simulink model "MATE_2level_DriveOversampling"  (R2024b)
settings: Solver=FixedStepDiscrete  StartTime=0.0  StopTime=1  FixedStep=Ts  MaxStep=10e-6  RelTol=1e-3
PostLoadFcn:
  | Ts=2e-6; Ts_Power=30e-6;
InitFcn:
  | Ts=2e-6; Ts_Power=30e-6;
libraries: simetranss x10, nesl_utility x9, fl_lib x6, ee_lib x6, batteryecm_lib x2, simulink x1
settings Model: ARTEMISmethode_block_infos=$$__separator__$$  ModifiedByFormat=x  Creator=Kyle  LastModifiedBy=x
settings SolverCC: AlgebraicLoopSolver=TrustRegion
settings DataIOCC: SaveFormat=Array  SignalLoggingSaveFormat=ModelDataLogs  SaveOutput=off  SignalLogging=off  SaveTime=off  ReturnWorkspaceOutputs=off
settings OptimizationCC: OptimizeBlockIOStorage=off  BufferReuse=off  GlobalBufferReuse=off  ExpressionFolding=off  ExpressionDepthLimit=2147483647  LocalBlockOutputs=off  InitFltsAndDblsToZero=on  LifeSpan=inf
settings DebuggingCC: SaveWithParameterizedLinksMsg=none  UnderspecifiedInitializationDetection=Classic  MergeDetectMultiDrivingBlocksExec=none  SignalResolutionControl=TryResolveAllWithWarning  SolverPrmCheckMsg=warning  MultiTaskDSMMsg=warning  MultiTaskCondExecSysMsg=none  FcnCallInpInsideContextMsg=warning  UnconnectedInputMsg=warning  UnconnectedOutputMsg=warning  UnconnectedLineMsg=warning  AllowSymbolicDim=off  StateNameClashWarn=warning  SFUnexpectedBacktrackingDiag=warning  SFNoUnconditionalDefaultTransitionDiag=warning  SFExecutionAtInitializationDiag=none  ArithmeticOperatorsInVariantConditions=warning
settings HardwareCC: ProdBitPerPointer=32  ProdBitPerSizeT=32  ProdBitPerPtrDiffT=32  ProdLargestAtomicFloat=None  ProdIntDivRoundTo=Undefined  ProdEndianess=Unspecified  ProdWordSize=32  ProdHWDeviceType=32-bit Generic  TargetHWDeviceType=32-bit Generic
settings ModelReferenceCC: EnableRefExpFcnMdlSchedulingChecks=on  PropagateSignalLabelsOutOfModel=off
settings SFSimCC: SimUseLocalCustomCode=off  CustomCodeUndefinedFunction=UseInterfaceOnly
settings RTWCC: RTWUseLocalCustomCode=off  GPUComputeCapability=3.5
settings CodeAppCC: StateflowObjectComments=on
settings GRTTargetCC: TargetFcnLib=ansi_tfl_tmw.mat  TargetLangStandard=C89/C90 (ANSI)  CombineOutputUpdateFcns=off  GRTInterface=on
settings ConfigComp: CovMetricSettings=dw  CovSaveCumulativeToWorkspaceVar=on  CovSaveSingleToWorkspaceVar=on  CovExternalEMLEnable=off
settings SimscapeCC: SimscapeNormalizeSystem=off

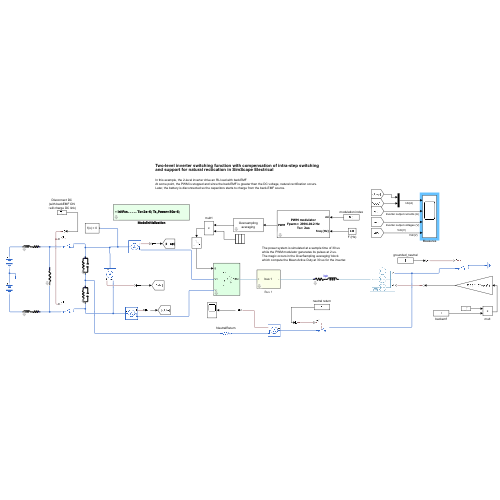
[thumbnail: Simulink's stored preview of the top-level diagram]
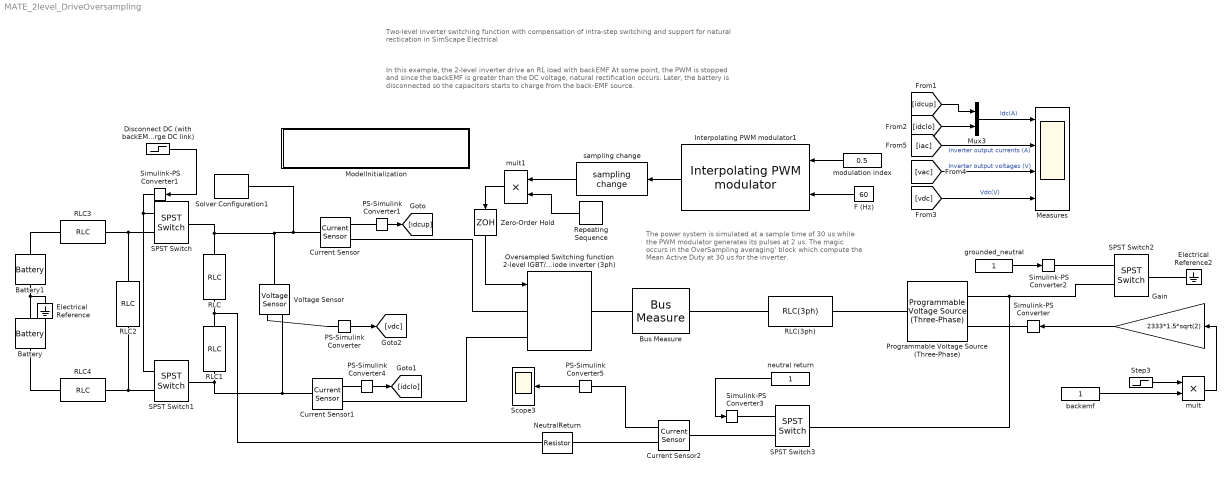
== system MATE_2level_DriveOversampling ==
  note: The power system is simulated at a sample time of 30 us
      | while the PWM modulator generates its pulses at 2 us.
      | The magic occurs in the OverSampling averaging' block
      | which compute the Mean Active Duty at 30 us for the inverter.
  note: In this example, the 2-level inverter drive an RL load with backEMF
      | At some point, the PWM is stopped and since the backEMF is greater than the DC voltage, natural rectification occurs.
      | Later, the battery is disconnected so the capacitors starts to charge from the back-EMF source.
  note: Two-level inverter switching function with compensation of intra-step switching
      | and support for natural rectication in SimScape Electrical
  Battery : batteryecm_lib/Battery  Vnom=2333 V  prm_dir=simscape.enum.battery.prm_dir.disabled  R1_dis=2 Ohm  R1_ch=2 Ohm  R1=0.001 Ohm  prm_AH=simscape.enum.battery.prm_AH.infinite  AH=50 A*hr  V1=11.5 V  AH1=25 A*hr  prm_R2=simscape.enum.battery.prm_R2.disabled  R2=2000 Ohm  Tmeas=298.15 K  charge_measurement_port=simscape.enum.battery.enable.no  prm_dyn=simscape.enum.battery.prm_dyn.off  Rp1=0.005 Ohm  tau1=30 s  Rp2=0.005 Ohm  tau2=30 s  Rp3=0.005 Ohm  tau3=30 s  Rp4=0.005 Ohm  tau4=30 s  Rp5=0.005 Ohm  tau5=30 s  prm_fade=simscape.enum.battery.prm_fade.disabled  N_fade=100  AH_fade=45 A*hr  R1_fade=2.02 Ohm  R1_ch_fade=2.02 Ohm  V1_fade=10.35 V  prm_age=simscape.enum.battery.prm_age.disabled  prm_age_OCV=simscape.enum.battery.prm_age_OCV.OCV  OCV_age=0.9  SOC_age=60  Tmeas_age=298.15 K  delta_time_age_vec=[0] d  temperature_age_vec=[273] K  OCV_scaling_age=2.2134e6  OCV_offset_age=1.632e6  temp_exp_age=0.515833569 V  t_exp_age=0.75  Vnom_T2=12 V  R1_T2=2.2 Ohm  R1_T2_dis=2.2 Ohm  R1_T2_ch=2.2 Ohm  V1_T2=11.4 V  R2_T2=2200 Ohm  Rp1_T2=0.005 Ohm  tau1_T2=30 s  Rp2_T2=0.005 Ohm  tau2_T2=30 s  Rp3_T2=0.005 Ohm  tau3_T2=30 s  Rp4_T2=0.005 Ohm  tau4_T2=30 s  Rp5_T2=0.005 Ohm  tau5_T2=30 s  Tmeas2=273.15 K  thermal_port=simscape.enum.thermaleffects.omit  thermal_mass=30000 J/K  i_specify=off  i_priority=None  i=0 A  i_nominal_specify=off  i_nominal_value=1  i_nominal_unit=A  v_specify=off  v_priority=None  v=0 V  v_nominal_specify=off  v_nominal_value=1  v_nominal_unit=V  charge_specify=off  charge_priority=High  charge=50 A*hr  charge_nominal_specify=off  charge_nominal_value=1  charge_nominal_unit=A*hr  num_cycles_specify=off  num_cycles_priority=High  num_cycles=0  num_cycles_nominal_specify=off  num_cycles_nominal_value=1  num_cycles_nominal_unit=1  temperature_specify=off  temperature_priority=High  temperature=298.15 K  temperature_nominal_specify=off  temperature_nominal_value=1  temperature_nominal_unit=K
  Battery1 : batteryecm_lib/Battery  Vnom=2333 V  prm_dir=simscape.enum.battery.prm_dir.disabled  R1_dis=2 Ohm  R1_ch=2 Ohm  R1=0.001 Ohm  prm_AH=simscape.enum.battery.prm_AH.infinite  AH=50 A*hr  V1=11.5 V  AH1=25 A*hr  prm_R2=simscape.enum.battery.prm_R2.disabled  R2=2000 Ohm  Tmeas=298.15 K  charge_measurement_port=simscape.enum.battery.enable.no  prm_dyn=simscape.enum.battery.prm_dyn.off  Rp1=0.005 Ohm  tau1=30 s  Rp2=0.005 Ohm  tau2=30 s  Rp3=0.005 Ohm  tau3=30 s  Rp4=0.005 Ohm  tau4=30 s  Rp5=0.005 Ohm  tau5=30 s  prm_fade=simscape.enum.battery.prm_fade.disabled  N_fade=100  AH_fade=45 A*hr  R1_fade=2.02 Ohm  R1_ch_fade=2.02 Ohm  V1_fade=10.35 V  prm_age=simscape.enum.battery.prm_age.disabled  prm_age_OCV=simscape.enum.battery.prm_age_OCV.OCV  OCV_age=0.9  SOC_age=60  Tmeas_age=298.15 K  delta_time_age_vec=[0] d  temperature_age_vec=[273] K  OCV_scaling_age=2.2134e6  OCV_offset_age=1.632e6  temp_exp_age=0.515833569 V  t_exp_age=0.75  Vnom_T2=12 V  R1_T2=2.2 Ohm  R1_T2_dis=2.2 Ohm  R1_T2_ch=2.2 Ohm  V1_T2=11.4 V  R2_T2=2200 Ohm  Rp1_T2=0.005 Ohm  tau1_T2=30 s  Rp2_T2=0.005 Ohm  tau2_T2=30 s  Rp3_T2=0.005 Ohm  tau3_T2=30 s  Rp4_T2=0.005 Ohm  tau4_T2=30 s  Rp5_T2=0.005 Ohm  tau5_T2=30 s  Tmeas2=273.15 K  thermal_port=simscape.enum.thermaleffects.omit  thermal_mass=30000 J/K  i_specify=off  i_priority=None  i=0 A  i_nominal_specify=off  i_nominal_value=1  i_nominal_unit=A  v_specify=off  v_priority=None  v=0 V  v_nominal_specify=off  v_nominal_value=1  v_nominal_unit=V  charge_specify=off  charge_priority=High  charge=50 A*hr  charge_nominal_specify=off  charge_nominal_value=1  charge_nominal_unit=A*hr  num_cycles_specify=off  num_cycles_priority=High  num_cycles=0  num_cycles_nominal_specify=off  num_cycles_nominal_value=1  num_cycles_nominal_unit=1  temperature_specify=off  temperature_priority=High  temperature=298.15 K  temperature_nominal_specify=off  temperature_nominal_value=1  temperature_nominal_unit=K
  Bus Measure : simetranss/Measure/Bus Measure  VoltageMeasurement=phase-to-ground  SetLabelV=on  LabelV=vac  Vpu=off  VpuLL=off  CurrentMeasurement=yes  SetLabelI=on  LabelI=iac  Ipu=off  Pbase=100e6  Vbase=500e3  bnumber=1  dis=off
      settings: AttributesFormatString=Bus %<bnumber>
  Current Sensor : fl_lib/Electrical/Electrical Sensors/Current Sensor
  Current Sensor1 : fl_lib/Electrical/Electrical Sensors/Current Sensor
  Current Sensor2 : fl_lib/Electrical/Electrical Sensors/Current Sensor
  "Disconnect DC (with backEMF ON : will charge DC link)" : Step  Time=0.6  Before=1  After=0  SampleTime=0
  Electrical Reference : fl_lib/Electrical/Electrical Elements/Electrical Reference
  Electrical Reference2 : fl_lib/Electrical/Electrical Elements/Electrical Reference
  F (Hz) : Constant  Value=60
  Gain : Gain  Gain=2333*1.5*sqrt(2)
  Interpolating PWM modulator1 : simetranss/Controllers/Interpolating PWM modulator  Tag=RTEcontrol_s38shd7k88  Fc=3000  Ts=Ts  Freq=60  Phase=0  Tdead=4e-4
  Measures : Scope  NumInputPorts=4
  ModelInitialization : Subsystem  mask(Model Functions){InitFcnX=Ts=2e-6; Ts_Power=30e-6;, prel=off, posl=on, inif=on, strf=off}
      mask prompts: InitFcnX "Initialisation"; prel "Preload Function"; posl "PostLoad Function"; inif "InitFcn"; strf "StartFcn"
      mask init:
      | if prel==1
      | 	set_param(bdroot, 'PreLoadFcn', InitFcnX);
      | else
      | 	set_param(bdroot, 'PreLoadFcn', '');
      | end
      | if inif==1
      | 	set_param(bdroot, 'InitFcn', InitFcnX);
      | else
      | 	set_param(bdroot, 'InitFcn', '');
      | end
      | if strf==1
      | 	set_param(bdroot, 'StartFcn', InitFcnX);
      | else
      | 	set_param(bdroot, 'StartFcn', '');
      | end
      | if posl==1
      | 	set_param(bdroot, 'PostLoadFcn', InitFcnX);
      | else
      | 	set_param(bdroot, 'PostLoadFcn', '');
      | end
      | PLF = get_param(bdroot, 'PreLoadFcn');
      | IF = get_param(bdroot, 'InitFcn');
      | SF = get_param(bdroot, 'StartFcn');
      | 
      | 
      | pos = get_param(gcb, 'Position');
      | width = pos(3) - pos(1); height = pos(4) - pos(2);
      mask Display:
      | text(5, height*0.5, [ ...
      |   ...
      | '- InitFcn. . . . . '  get_param(bdroot, 'InitFcn')  ...
      | ], ...
      | 'horizontalAlignment', 'left', 'verticalAlignment', 'middle') ;
  Mux3 : Mux  Inputs=2
  NeutralReturn : ee_lib/Passive/Resistor  R=1e-4 Ohm  enable_R_tol=ee.enum.toleranceApplication.none  R_tol=5  tol_distribution=ee.enum.toleranceDistribution.uniform  nSigma=4  enable_operating_limits=ee.enum.enable.no  operating_limit_action=ee.enum.passive.reportOpLim.warn  power_rating=1 W  max_working_voltage=100 V  noise_mode=ee.enum.sources.noise.Disabled  Tdevice=25 degC  sample_time=1e-3 s  repeatability=ee.enum.ic.repeatability.notRepeatable  user_seed=0  auto_seed=415452298  fault_action=simscape.enum.assert.action.none  t_fault=1 s  power_derating_T1=70 degC  power_derating_T2=155 degC  operating_temperature_range_vec=[-50, 150] degC  alpha=3.93e-3 1/K  Tmeas=25 degC  thermal_mass=100 J/K  temperature_specify=off  temperature_priority=High  temperature=298.15 K  temperature_nominal_specify=off  temperature_nominal_value=1  temperature_nominal_unit=K
  Oversampled Switching function 2-level IGBT/diode inverter (3ph) : simetranss/Power converters/Oversampled Switching function 2-level IGBT//diode inverter (3ph)  Ron=1e-3  Rsnubber=100  Csnubber=1e-6  Vf=1  Ts=Ts_Power
  PS-Simulink Converter{,1,4..5} (4 alike) : nesl_utility/PS-Simulink Converter  PhysicalDomain=network_engine_domain  SubClassName=ps_output  LeftPortType=input  RightPortType=output  PseudoPeriodic=off  Frequencies=[]  VectorFormat=inherit  Unit=inherit  AffineConversion=off
  Programmable Voltage Source (Three-Phase) : ee_lib/Sources/Programmable Voltage Source (Three-Phase)  magnitude_type=ee.enum.timechanging.external  vline_rms=100 V  magn_ramp=1 V/s  magn_step=1 V  magn_modu_magn=1 V  magn_modu_freq=1 Hz  magn_t1=1 s  magn_t2=2 s  frequency_type=ee.enum.timechanging.constant  freq=60 Hz  freq_ramp=1 Hz/s  freq_step=1 Hz  freq_modu_magn=1 Hz  freq_modu_freq=1 Hz  freq_t1=1 s  freq_t2=2 s  phase_type=ee.enum.timechanging.constant  shift=0 deg  phase_ramp=1 deg/s  phase_step=1 deg  phase_modu_magn=1 deg  phase_modu_freq=1 Hz  phase_t1=1 s  phase_t2=2 s  impedance_option=1  SShortCircuit=1e6 A*V  XR=15  R=0.01 Ohm  L=3.97e-4 H  G_parasitic=1e-6 1/Ohm  harmonic_option=0  harmonic_orders=[5, 7, 11, 13]  harmonic_ratios=[.1, .1, .1, .1]  harmonic_shifts=[0, 0, 0, 0] deg  harmonic_sequences=[1, 1, 1, 1]  harmonic_t1=-inf s  harmonic_t2=inf s  I_specify=off  I_priority=None  I=[0, 0, 0] A  I_nominal_specify=off  I_nominal_value=1  I_nominal_unit=A  V_specify=off  V_priority=None  V=[0, 0, 0] V  V_nominal_specify=off  V_nominal_value=1  V_nominal_unit=V
      settings: InternalSimscapePortConfiguration="{\"Bottom\":[],\"Left\":[{\"id\":\"ext_magn\",\"label\":\"M\",\"type\":\"input\"},{\"id\":\"n\",\"label\":\"n\",\"type\":\"foundation.electrical.electrical\"}],\"Right\":[{\"id\":\"N\",\"label\":\"~\",\"type\":\"foundation.electrical.three_phase\"}],\"Top\":[]}"
  RLC : simetranss/Passive/RLC  BranchType=RC  SerPar=Parallel  Resistance=4e3  Inductance=1e-3  Capacitance=10e-3  Ropen=1e9
  RLC(3ph) : simetranss/Passive/RLC(3ph)  BranchType=RL  SerPar=Series  Resistance=5  Inductance=10e-3  Capacitance=1e-6  Ropen=1e9
  RLC1 : simetranss/Passive/RLC  BranchType=RC  SerPar=Parallel  Resistance=4e3  Inductance=1e-3  Capacitance=10e-3  Ropen=1e9
  RLC2 : simetranss/Passive/RLC  BranchType=R  SerPar=Parallel  Resistance=50e3  Inductance=1e-3  Capacitance=10e-3  Ropen=1e9
  RLC3 : simetranss/Passive/RLC  BranchType=RL  SerPar=Series  Resistance=0.003  Inductance=1e-4  Capacitance=10e-3  Ropen=1e9
  RLC4 : simetranss/Passive/RLC  BranchType=RL  SerPar=Series  Resistance=0.003  Inductance=1e-4  Capacitance=10e-3  Ropen=1e9
  Repeating Sequence : simulink/Sources/Repeating Sequence  rep_seq_t="[0 0.1 0.1+Ts  0.4 0.4+Ts 10]"  rep_seq_y="[0  0  1            1     0       0]"
  SPST Switch : ee_lib/Switches & Breakers/SPST Switch  R_closed=1e-3 Ohm  G_open=1e-6 S  Threshold=0.5 V  Width=0 V  model_dynamics=0  t_on=1e-3 s  t_off=1e-3 s  initial_vT=0 V
      settings: InternalSimscapePortConfiguration="{\"Bottom\":[],\"Left\":[{\"id\":\"vT\",\"label\":\"vT\",\"type\":\"input\"},{\"id\":\"p\",\"label\":\"\",\"type\":\"foundation.electrical.electrical\"}],\"Right\":[{\"id\":\"n\",\"label\":\"\",\"type\":\"foundation.electrical.electrical\"}],\"Top\":[]}"
  SPST Switch1 : ee_lib/Switches & Breakers/SPST Switch  R_closed=1e-3 Ohm  G_open=1e-6 S  Threshold=0.5 V  Width=0 V  model_dynamics=0  t_on=1e-3 s  t_off=1e-3 s  initial_vT=0 V
      settings: InternalSimscapePortConfiguration="{\"Bottom\":[],\"Left\":[{\"id\":\"vT\",\"label\":\"vT\",\"type\":\"input\"},{\"id\":\"p\",\"label\":\"\",\"type\":\"foundation.electrical.electrical\"}],\"Right\":[{\"id\":\"n\",\"label\":\"\",\"type\":\"foundation.electrical.electrical\"}],\"Top\":[]}"
  SPST Switch2 : ee_lib/Switches & Breakers/SPST Switch  R_closed=1e-3 Ohm  G_open=1e-4 S  Threshold=0.5 V  Width=0 V  model_dynamics=0  t_on=1e-3 s  t_off=1e-3 s  initial_vT=0 V
      settings: InternalSimscapePortConfiguration="{\"Bottom\":[],\"Left\":[{\"id\":\"vT\",\"label\":\"vT\",\"type\":\"input\"},{\"id\":\"p\",\"label\":\"\",\"type\":\"foundation.electrical.electrical\"}],\"Right\":[{\"id\":\"n\",\"label\":\"\",\"type\":\"foundation.electrical.electrical\"}],\"Top\":[]}"
  SPST Switch3 : ee_lib/Switches & Breakers/SPST Switch  R_closed=1e-3 Ohm  G_open=1e-6 S  Threshold=0.5 V  Width=0 V  model_dynamics=0  t_on=1e-3 s  t_off=1e-3 s  initial_vT=0 V
      settings: InternalSimscapePortConfiguration="{\"Bottom\":[],\"Left\":[{\"id\":\"vT\",\"label\":\"vT\",\"type\":\"input\"},{\"id\":\"p\",\"label\":\"\",\"type\":\"foundation.electrical.electrical\"}],\"Right\":[{\"id\":\"n\",\"label\":\"\",\"type\":\"foundation.electrical.electrical\"}],\"Top\":[]}"
  Scope3 : Scope
  Simulink-PS Converter{,1..3} (4 alike) : nesl_utility/Simulink-PS Converter  PhysicalDomain=network_engine_domain  SubClassName=ps_input  LeftPortType=input  RightPortType=output  PseudoPeriodic=off  Frequencies=[]  NoiseDistribution=none  NoiseParameters=[]  Unit=1  AffineConversion=off  FilteringAndDerivatives=provide  SimscapeFilterOrder=1  InputFilterTimeConstant=0.001  UdotUserProvided=0
  Solver Configuration1 : nesl_utility/Solver Configuration  PhysicalDomain=network_engine_domain  SubClassName=solver  LeftPortType=input  RightPortType=generic  Tones=[]  Harmonics=[]  SimulateNoise=off  Profile=off  UseLocalSampling=off  EnableSwitchedLinearOptims=on  FrequencyDomain=off  UseCCode=off  RelTol=0.001  AbsTol=1e-06  MinStep=1e-09  ToWorkspace=off  RevertToSquareIcSolve=off  NumHomotopyIterations=100  PhasorMode=off  PhasorModeNumHarmonics=1  ConsistencySolver=NEWTON_FTOL  IndexReductionMethod=DerivativeReplacement  DoDC=off  ResidualTolerance=0.001  ConsistencyTolSource=GLOBAL  ConsistencyAbsTol=0.001  ConsistencyRelTol=0.001  ConsistencyTolFactor=0.001  UseLocalSolver=on  LocalSolverChoice=NE_PARTITIONING_ADVANCER  ResolveIndetEquations=off  FunctionEvalNumThread=1  LocalSolverSampleTime=Ts_Power  DoFixedCost=on  MaxNonlinIter=1  MaxModeIter=2  ComputeImpulses=off  ImpulseIterations=2  LinearAlgebra=Sparse  LinearAlgebraNumThread=0  EquationFormulation=NE_TIME_EF  DelaysMemoryBudget=1024  AutomaticFiltering=off  FilteringTimeConstant=0.001  PartitionStorageMethod=AS_NEEDED  PartitionMemoryBudget=1024  PartitionMethod=ROBUST  MultibodyUseLocalSolver=off  MultibodyLocalSolverChoice=ODE1  MultibodyLocalSolverSampleTime=0.001
  Step3 : Step  Time=0.08  SampleTime=0
  Voltage Sensor : fl_lib/Electrical/Electrical Sensors/Voltage Sensor
  Zero-Order Hold : ZeroOrderHold  SampleTime=Ts_Power
  backemf : Constant
  grounded_neutral : Constant
  modulation index : Constant  Value=0.5
  mult : Product
  mult1 : Product
  neutral return : Constant
  sampling change : simetranss/Controllers/sampling change  rate=100  Ts=Ts
  wires:
  "Disconnect DC (with backEMF ON : will charge DC link)"/1 -> Simulink-PS Converter1/1
  Gain/1 -> Simulink-PS Converter/1
  F (Hz)/1 -> Interpolating PWM modulator1/2
  modulation index/1 -> Interpolating PWM modulator1/1
  mult1/1 -> Zero-Order Hold/1
  Repeating Sequence/1 -> mult1/2
  neutral return/1 -> Simulink-PS Converter3/1
  backemf/1 -> mult/2
  mult/1 -> Gain/1
  Step3/1 -> mult/1
  [vdc] -> Measures/4  "Vdc(V)"
  grounded_neutral/1 -> Simulink-PS Converter2/1
  Mux3/1 -> Measures/1  "Idc(A)"
  PS-Simulink Converter5/1 -> Scope3/1
  PS-Simulink Converter1/1 -> [idcup]
  PS-Simulink Converter/1 -> [vdc]
  [idcup] -> Mux3/1
  [idclo] -> Mux3/2
  [iac] -> Measures/2  "Inverter output currents (A)"
  [vac] -> Measures/3  "Inverter output voltages (V)"
  Interpolating PWM modulator1/1 -> sampling change/1
  Zero-Order Hold/1 -> Oversampled Switching function 2-level IGBT/diode inverter (3ph)/1
  sampling change/1 -> mult1/1
  PS-Simulink Converter4/1 -> [idclo]
  connections:
  Simulink-PS Converter1/RConn1 -- SPST Switch1/LConn1 -- SPST Switch/LConn1
  Current Sensor1/RConn1 -- PS-Simulink Converter4/LConn1
  Simulink-PS Converter/RConn1 -- Programmable Voltage Source (Three-Phase)/LConn1
  Programmable Voltage Source (Three-Phase)/LConn2 -- SPST Switch2/LConn2 -- SPST Switch3/RConn1
  Oversampled Switching function 2-level IGBT/diode inverter (3ph)/LConn1 -- Current Sensor/RConn2
  PS-Simulink Converter1/LConn1 -- Current Sensor/RConn1
  PS-Simulink Converter/LConn1 -- Voltage Sensor/RConn1
  SPST Switch1/RConn1 -- Voltage Sensor/RConn2 -- Current Sensor1/LConn1 -- RLC1/RConn1
  SPST Switch/RConn1 -- RLC/LConn1 -- Voltage Sensor/LConn1 -- Solver Configuration1/RConn1 -- Current Sensor/LConn1
  RLC2/RConn1 -- RLC4/LConn1 -- SPST Switch1/LConn2
  SPST Switch/LConn2 -- RLC2/LConn1 -- RLC3/LConn1
  RLC4/RConn1 -- Battery/RConn1
  RLC3/RConn1 -- Battery1/LConn1
  Battery/LConn1 -- Electrical Reference/LConn1 -- Battery1/RConn1
  RLC/RConn1 -- RLC1/LConn1 -- NeutralReturn/RConn1
  RLC(3ph)/LConn1 -- Bus Measure/RConn1
  RLC(3ph)/RConn1 -- Programmable Voltage Source (Three-Phase)/RConn1
  Bus Measure/LConn1 -- Oversampled Switching function 2-level IGBT/diode inverter (3ph)/RConn1
  SPST Switch2/RConn1 -- Electrical Reference2/LConn1
  Simulink-PS Converter2/RConn1 -- SPST Switch2/LConn1
  Current Sensor2/RConn2 -- NeutralReturn/LConn1
  SPST Switch3/LConn2 -- Current Sensor2/LConn1
  Simulink-PS Converter3/RConn1 -- SPST Switch3/LConn1
  Current Sensor2/RConn1 -- PS-Simulink Converter5/LConn1
  Current Sensor1/RConn2 -- Oversampled Switching function 2-level IGBT/diode inverter (3ph)/LConn2

== system MATE_2level_DriveOversampling/ModelInitialization ==
